simulink model "My_gfm_battery_sil_2_Exciter_Dis"  (R2018b)
settings: Solver=ode4  StartTime=0.0  StopTime=5  MaxStep=1e-4  RelTol=1e-3
PreLoadFcn:
  | modelDir = fileparts(get_param(bdroot,'FileName'));
  | 
  | load_system(fullfile(modelDir,'controls_element_lib.slx'));
  | load_system(fullfile(modelDir,'test_sequence_lib.slx'));
InitFcn:
  | close all;
  | clear all;
  | clc;
  | 
  | Ts_Power = 50e-6;
  | 
  | % frequency nominals
  | F_NOM = 60;
  | W_NOM = 2 * pi * F_NOM;
  | 
  | % base values relative to inverter
  | % --------------------------------
  | VLL_INV_NOM = 480;
  | P_INV_NOM = 1e6;
  | Q_INV_NOM = 0.5e6;
  | S_INV_NOM = sqrt(P_INV_NOM^2 + Q_INV_NOM^2);
  | 
  | I_INV_BASE = S_INV_NOM/(sqrt(3)*VLL_INV_NOM);
  | Z_INV_BASE = VLL_INV_NOM^2/S_INV_NOM;
  | L_INV_BASE = Z_INV_BASE / W_NOM;
  | C_INV_BASE = 1 / (Z_INV_BASE * W_NOM);
  | 
  | % nominal ratings for power system model
  | % --------------------------------------
  | INVERTER_COUNT = 100;
  | 
  | VLV_NOM = VLL_INV_NOM;
  | VMV_NOM = 35e3;
  | VHV_NOM = 230e3;
  | S_PLANT = INVERTER_COUNT * S_INV_NOM;
  | 
  | N_GSU = VHV_NOM/VMV_NOM;
  | N_MVT = VMV_NOM/VLV_NOM;
  | 
  | I_LV_BASE = S_PLANT/(sqrt(3)*VLV_NOM);
  | I_MV_BASE = S_PLANT/(sqrt(3)*VMV_NOM);
  | I_HV_BASE = S_PLANT/(sqrt(3)*VHV_NOM);
  | 
  | Z_LV_BASE = VLV_NOM^2/S_PLANT;
  | Z_MV_BASE = VMV_NOM^2/S_PLANT;
  | Z_HV_BASE = VHV_NOM^2/S_PLANT;
  | 
  | L_LV_BASE = Z_LV_BASE / W_NOM;
  | L_MV_BASE = Z_MV_BASE / W_NOM;
  | L_HV_BASE = Z_HV_BASE / W_NOM;
  | C_LV_BASE = 1 / (Z_LV_BASE * W_NOM);
  | C_MV_BASE = 1 / (Z_MV_BASE * W_NOM);
  | C_HV_BASE = 1 / (Z_HV_BASE * W_NOM);
undefined symbols (not defined in the file): DiscIntNeverNeededParam, j
libraries: simulink x27, test_sequence_lib x10, controls_element_lib x3
(part 4 of 5)

== system My_gfm_battery_sil_2_Exciter_Dis/My Inverter Controller /My_circuit_controls_A1/LPF1 ==
  note: Forward integrator
  in : Inport
  Constant2 : Constant  Value=Ts
  Constant3 : Constant  Value=OmegaUp
  Constant4 : Constant  Value=OmegaDn
  Constant9 : Constant  Value=1/20000
  Delay : Delay  DelayLength=1  InitialCondition=0
  Gain : Gain  Gain=1/5
  Math Function : Math  Operator=reciprocal  SaturateOnIntegerOverflow=on
  MinMax : MinMax  Function=max  Inputs=2
  MinMax1 : MinMax  Inputs=2
  MinMax2 : MinMax  Inputs=2
  Product : Product
  Product1 : Product
  Product2 : Product
  Saturation : Saturate  UpperLimit=inf  LowerLimit=0
  Saturation1 : Saturate  UpperLimit=0  LowerLimit=-inf
  Sum : Sum  Inputs=|++
  Sum1 : Sum  Inputs=|++
  Sum4 : Sum  Inputs=|+-
  out : Outport  VectorParamsAs1DForOutWhenUnconnected=on
  wires:
  Delay/1 -> out/1, Sum4/2, Sum/2
  in/1 -> Sum4/1
  Sum4/1 -> Product2/1, Product1/2
  Sum/1 -> Delay/1
  Saturation/1 -> Sum1/1
  Saturation1/1 -> Sum1/2
  Sum1/1 -> Product/2
  Product/1 -> Sum/1
  [Ts] -> Product/1
  [OmegaUp] -> Product1/1
  [OmegaDn] -> Product2/2
  Constant2/1 -> MinMax/1
  MinMax/1 -> [Ts]
  Constant9/1 -> MinMax/2
  MinMax1/1 -> [OmegaUp]
  MinMax2/1 -> [OmegaDn]
  [Ts] -> Math Function/1
  Math Function/1 -> Gain/1
  Gain/1 -> MinMax1/2, MinMax2/1
  Constant3/1 -> MinMax1/1
  Constant4/1 -> MinMax2/2
  Product1/1 -> Saturation/1
  Product2/1 -> Saturation1/1

== system My_gfm_battery_sil_2_Exciter_Dis/My Inverter Controller /My_circuit_controls_A1/LPF2 ==
  1 : Inport
  Gain2 : Gain  Gain=1/20e-6
  Integrator : Integrator
  Sum4 : Sum  Inputs=|+-
  Out1 : Outport  VectorParamsAs1DForOutWhenUnconnected=on
  wires:
  Sum4/1 -> Gain2/1
  1/1 -> Sum4/1
  Integrator/1 -> Out1/1, Sum4/2
  Gain2/1 -> Integrator/1

== system My_gfm_battery_sil_2_Exciter_Dis/My Inverter Controller /My_circuit_controls_A1/LPF3 ==
  note: Forward integrator
  in : Inport
  Constant2 : Constant  Value=Ts
  Constant3 : Constant  Value=OmegaUp
  Constant4 : Constant  Value=OmegaDn
  Constant9 : Constant  Value=1/20000
  Delay : Delay  DelayLength=1  InitialCondition=0
  Gain : Gain  Gain=1/5
  Math Function : Math  Operator=reciprocal  SaturateOnIntegerOverflow=on
  MinMax : MinMax  Function=max  Inputs=2
  MinMax1 : MinMax  Inputs=2
  MinMax2 : MinMax  Inputs=2
  Product : Product
  Product1 : Product
  Product2 : Product
  Saturation : Saturate  UpperLimit=inf  LowerLimit=0
  Saturation1 : Saturate  UpperLimit=0  LowerLimit=-inf
  Sum : Sum  Inputs=|++
  Sum1 : Sum  Inputs=|++
  Sum4 : Sum  Inputs=|+-
  out : Outport  VectorParamsAs1DForOutWhenUnconnected=on
  wires:
  Delay/1 -> out/1, Sum4/2, Sum/2
  in/1 -> Sum4/1
  Sum4/1 -> Product2/1, Product1/2
  Sum/1 -> Delay/1
  Saturation/1 -> Sum1/1
  Saturation1/1 -> Sum1/2
  Sum1/1 -> Product/2
  Product/1 -> Sum/1
  [Ts] -> Product/1
  [OmegaUp] -> Product1/1
  [OmegaDn] -> Product2/2
  Constant2/1 -> MinMax/1
  MinMax/1 -> [Ts]
  Constant9/1 -> MinMax/2
  MinMax1/1 -> [OmegaUp]
  MinMax2/1 -> [OmegaDn]
  [Ts] -> Math Function/1
  Math Function/1 -> Gain/1
  Gain/1 -> MinMax1/2, MinMax2/1
  Constant3/1 -> MinMax1/1
  Constant4/1 -> MinMax2/2
  Product1/1 -> Saturation/1
  Product2/1 -> Saturation1/1

== system My_gfm_battery_sil_2_Exciter_Dis/My Inverter Controller /My_circuit_controls_A1/LPF4 ==
  note: Forward integrator
  in : Inport
  Constant2 : Constant  Value=Ts
  Constant3 : Constant  Value=OmegaUp
  Constant4 : Constant  Value=OmegaDn
  Constant9 : Constant  Value=1/20000
  Delay : Delay  DelayLength=1  InitialCondition=0
  Gain : Gain  Gain=1/5
  Math Function : Math  Operator=reciprocal  SaturateOnIntegerOverflow=on
  MinMax : MinMax  Function=max  Inputs=2
  MinMax1 : MinMax  Inputs=2
  MinMax2 : MinMax  Inputs=2
  Product : Product
  Product1 : Product
  Product2 : Product
  Saturation : Saturate  UpperLimit=inf  LowerLimit=0
  Saturation1 : Saturate  UpperLimit=0  LowerLimit=-inf
  Sum : Sum  Inputs=|++
  Sum1 : Sum  Inputs=|++
  Sum4 : Sum  Inputs=|+-
  out : Outport  VectorParamsAs1DForOutWhenUnconnected=on
  wires:
  Delay/1 -> out/1, Sum4/2, Sum/2
  in/1 -> Sum4/1
  Sum4/1 -> Product2/1, Product1/2
  Sum/1 -> Delay/1
  Saturation/1 -> Sum1/1
  Saturation1/1 -> Sum1/2
  Sum1/1 -> Product/2
  Product/1 -> Sum/1
  [Ts] -> Product/1
  [OmegaUp] -> Product1/1
  [OmegaDn] -> Product2/2
  Constant2/1 -> MinMax/1
  MinMax/1 -> [Ts]
  Constant9/1 -> MinMax/2
  MinMax1/1 -> [OmegaUp]
  MinMax2/1 -> [OmegaDn]
  [Ts] -> Math Function/1
  Math Function/1 -> Gain/1
  Gain/1 -> MinMax1/2, MinMax2/1
  Constant3/1 -> MinMax1/1
  Constant4/1 -> MinMax2/2
  Product1/1 -> Saturation/1
  Product2/1 -> Saturation1/1

== system My_gfm_battery_sil_2_Exciter_Dis/My Inverter Controller /My_circuit_controls_A1/SOGI ==
  in : Inport
  f : Inport  Port=2
  Constant2 : Constant  Value=Ts
  Constant9 : Constant  Value=1/20000
  Gain : Gain
  Gain2 : Gain  Gain=2*pi
  Integrator1 : Subsystem
  Integrator3 : Subsystem
  MinMax : MinMax  Function=max  Inputs=2
  Product : Product
  Product2 : Product
  Sum : Sum  Inputs=|+-
  Sum1 : Sum  Inputs=|+-
  Notched : Outport  VectorParamsAs1DForOutWhenUnconnected=on
  BandPassed : Outport  Port=2  VectorParamsAs1DForOutWhenUnconnected=on
  wires:
  f/1 -> Gain2/1
  in/1 -> Sum1/1
  Integrator1/1(Out) -> Product2/1
  Gain/1 -> Sum1/2
  Sum1/1 -> Notched/1, Sum/1
  Integrator3/1(Out) -> Gain/1, BandPassed/1, Integrator1/1(In)
  Gain2/1 -> Product2/2, Product/2
  Sum/1 -> Product/1
  Product2/1 -> Sum/2
  [Ts] -> Integrator3/2(Ts)
  Product/1 -> Integrator3/1(In)
  [Ts] -> Integrator1/2(Ts)
  MinMax/1 -> [Ts]
  Constant2/1 -> MinMax/1
  Constant9/1 -> MinMax/2

== system My_gfm_battery_sil_2_Exciter_Dis/My Inverter Controller /My_circuit_controls_A1/virtual damper ==
  v : Inport
  Damping HPF : Subsystem  mask(High Pass Filter){Ts=1/20000, OmegaUp=1/250e-6, OmegaDn=1/250e-6}
      mask prompts: Ts "Tsample"; OmegaUp "Up Path Bandwidth"; OmegaDn "Down Path Bandwidth"
      mask help: Min. Tsample is 1/20000; Max. Omega is 0.2/Ts
      mask DialogControl Container2 Prompt: Parameters
  g_damp : Gain  Gain=1/(0.8*Z_INV_BASE)
  i_damp : Outport  VectorParamsAs1DForOutWhenUnconnected=on
  wires:
  g_damp/1 -> i_damp/1
  v/1 -> Damping HPF/1(in)
  Damping HPF/1(out) -> g_damp/1

== system My_gfm_battery_sil_2_Exciter_Dis/My Inverter Controller /My_circuit_controls_A2/LPF ==
  1 : Inport
  Gain2 : Gain  Gain=1/20e-6
  Integrator : Integrator
  Sum4 : Sum  Inputs=|+-
  Out1 : Outport  VectorParamsAs1DForOutWhenUnconnected=on
  wires:
  Gain2/1 -> Integrator/1
  Integrator/1 -> Sum4/2, Out1/1
  1/1 -> Sum4/1
  Sum4/1 -> Gain2/1

== system My_gfm_battery_sil_2_Exciter_Dis/My Inverter Controller /My_circuit_controls_A2/LPF1 ==
  1 : Inport
  Gain2 : Gain  Gain=1/20e-6
  Integrator : Integrator
  Sum4 : Sum  Inputs=|+-
  Out1 : Outport  VectorParamsAs1DForOutWhenUnconnected=on
  wires:
  Gain2/1 -> Integrator/1
  Integrator/1 -> Sum4/2, Out1/1
  1/1 -> Sum4/1
  Sum4/1 -> Gain2/1

== system My_gfm_battery_sil_2_Exciter_Dis/My Inverter Controller /My_circuit_controls_A2/LPF2 ==
  1 : Inport
  Gain2 : Gain  Gain=1/20e-6
  Integrator : Integrator
  Sum4 : Sum  Inputs=|+-
  Out1 : Outport  VectorParamsAs1DForOutWhenUnconnected=on
  wires:
  Sum4/1 -> Gain2/1
  1/1 -> Sum4/1
  Integrator/1 -> Out1/1, Sum4/2
  Gain2/1 -> Integrator/1

== system My_gfm_battery_sil_2_Exciter_Dis/My Inverter Controller /My_circuit_controls_A2/LPF3 ==
  1 : Inport
  Gain2 : Gain  Gain=1/500e-6
  Integrator : Integrator
  Sum4 : Sum  Inputs=|+-
  Out1 : Outport  VectorParamsAs1DForOutWhenUnconnected=on
  wires:
  Gain2/1 -> Integrator/1
  Integrator/1 -> Sum4/2, Out1/1
  1/1 -> Sum4/1
  Sum4/1 -> Gain2/1

== system My_gfm_battery_sil_2_Exciter_Dis/My Inverter Controller /My_circuit_controls_A2/LPF4 ==
  1 : Inport
  Gain2 : Gain  Gain=1/20e-6
  Integrator : Integrator
  Sum4 : Sum  Inputs=|+-
  Out1 : Outport  VectorParamsAs1DForOutWhenUnconnected=on
  wires:
  Gain2/1 -> Integrator/1
  Integrator/1 -> Sum4/2, Out1/1
  1/1 -> Sum4/1
  Sum4/1 -> Gain2/1

== system My_gfm_battery_sil_2_Exciter_Dis/My Inverter Controller /My_circuit_controls_A2/SOGI_BPF ==
  in : Inport
  f : Inport  Port=2
  Gain : Gain
  Gain2 : Gain  Gain=2*pi
  Integrator : Integrator
  Integrator1 : Integrator
  Product : Product
  Product2 : Product
  Sum : Sum  Inputs=|+-
  Sum1 : Sum  Inputs=|+-
  Notched : Outport  VectorParamsAs1DForOutWhenUnconnected=on
  wires:
  f/1 -> Gain2/1
  in/1 -> Sum1/1
  Product/1 -> Integrator/1
  Integrator1/1 -> Product2/1
  Gain/1 -> Sum1/2
  Sum1/1 -> Notched/1, Sum/1
  Integrator/1 -> Integrator1/1, Gain/1
  Gain2/1 -> Product2/2, Product/2
  Sum/1 -> Product/1
  Product2/1 -> Sum/2

== system My_gfm_battery_sil_2_Exciter_Dis/My Inverter Controller /My_circuit_controls_A2/virtual damper ==
  v : Inport
  1/tau_damp : Gain  Gain=1/250e-6
  Integrator : Integrator
  Sum : Sum  Inputs=|+-
  g_damp : Gain  Gain=1/(0.8*Z_INV_BASE)
  i_damp : Outport  VectorParamsAs1DForOutWhenUnconnected=on
  wires:
  g_damp/1 -> i_damp/1
  Sum/1 -> g_damp/1, 1/tau_damp/1
  v/1 -> Sum/1
  1/tau_damp/1 -> Integrator/1
  Integrator/1 -> Sum/2

== system My_gfm_battery_sil_2_Exciter_Dis/My Inverter Controller /My_circuit_controls_A3/LPF ==
  1 : Inport
  Gain2 : Gain  Gain=1/20e-6
  Integrator : Integrator
  Sum4 : Sum  Inputs=|+-
  Out1 : Outport  VectorParamsAs1DForOutWhenUnconnected=on
  wires:
  Gain2/1 -> Integrator/1
  Integrator/1 -> Sum4/2, Out1/1
  1/1 -> Sum4/1
  Sum4/1 -> Gain2/1

== system My_gfm_battery_sil_2_Exciter_Dis/My Inverter Controller /My_circuit_controls_A3/LPF1 ==
  1 : Inport
  Gain2 : Gain  Gain=1/20e-6
  Integrator : Integrator
  Sum4 : Sum  Inputs=|+-
  Out1 : Outport  VectorParamsAs1DForOutWhenUnconnected=on
  wires:
  Gain2/1 -> Integrator/1
  Integrator/1 -> Sum4/2, Out1/1
  1/1 -> Sum4/1
  Sum4/1 -> Gain2/1

== system My_gfm_battery_sil_2_Exciter_Dis/My Inverter Controller /My_circuit_controls_A3/LPF2 ==
  1 : Inport
  Gain2 : Gain  Gain=1/20e-6
  Integrator : Integrator
  Sum4 : Sum  Inputs=|+-
  Out1 : Outport  VectorParamsAs1DForOutWhenUnconnected=on
  wires:
  Sum4/1 -> Gain2/1
  1/1 -> Sum4/1
  Integrator/1 -> Out1/1, Sum4/2
  Gain2/1 -> Integrator/1

== system My_gfm_battery_sil_2_Exciter_Dis/My Inverter Controller /My_circuit_controls_A3/LPF3 ==
  note: Forward integrator
  in : Inport
  Constant2 : Constant  Value=Ts
  Constant3 : Constant  Value=OmegaUp
  Constant4 : Constant  Value=OmegaDn
  Constant9 : Constant  Value=1/20000
  Delay : Delay  DelayLength=1  InitialCondition=0
  Gain : Gain  Gain=1/5
  Math Function : Math  Operator=reciprocal  SaturateOnIntegerOverflow=on
  MinMax : MinMax  Function=max  Inputs=2
  MinMax1 : MinMax  Inputs=2
  MinMax2 : MinMax  Inputs=2
  Product : Product
  Product1 : Product
  Product2 : Product
  Saturation : Saturate  UpperLimit=inf  LowerLimit=0
  Saturation1 : Saturate  UpperLimit=0  LowerLimit=-inf
  Sum : Sum  Inputs=|++
  Sum1 : Sum  Inputs=|++
  Sum4 : Sum  Inputs=|+-
  out : Outport  VectorParamsAs1DForOutWhenUnconnected=on
  wires:
  Delay/1 -> out/1, Sum4/2, Sum/2
  in/1 -> Sum4/1
  Sum4/1 -> Product2/1, Product1/2
  Sum/1 -> Delay/1
  Saturation/1 -> Sum1/1
  Saturation1/1 -> Sum1/2
  Sum1/1 -> Product/2
  Product/1 -> Sum/1
  [Ts] -> Product/1
  [OmegaUp] -> Product1/1
  [OmegaDn] -> Product2/2
  Constant2/1 -> MinMax/1
  MinMax/1 -> [Ts]
  Constant9/1 -> MinMax/2
  MinMax1/1 -> [OmegaUp]
  MinMax2/1 -> [OmegaDn]
  [Ts] -> Math Function/1
  Math Function/1 -> Gain/1
  Gain/1 -> MinMax1/2, MinMax2/1
  Constant3/1 -> MinMax1/1
  Constant4/1 -> MinMax2/2
  Product1/1 -> Saturation/1
  Product2/1 -> Saturation1/1

== system My_gfm_battery_sil_2_Exciter_Dis/My Inverter Controller /My_circuit_controls_A3/LPF4 ==
  note: Forward integrator
  in : Inport
  Constant2 : Constant  Value=Ts
  Constant3 : Constant  Value=OmegaUp
  Constant4 : Constant  Value=OmegaDn
  Constant9 : Constant  Value=1/20000
  Delay : Delay  DelayLength=1  InitialCondition=0
  Gain : Gain  Gain=1/5
  Math Function : Math  Operator=reciprocal  SaturateOnIntegerOverflow=on
  MinMax : MinMax  Function=max  Inputs=2
  MinMax1 : MinMax  Inputs=2
  MinMax2 : MinMax  Inputs=2
  Product : Product
  Product1 : Product
  Product2 : Product
  Saturation : Saturate  UpperLimit=inf  LowerLimit=0
  Saturation1 : Saturate  UpperLimit=0  LowerLimit=-inf
  Sum : Sum  Inputs=|++
  Sum1 : Sum  Inputs=|++
  Sum4 : Sum  Inputs=|+-
  out : Outport  VectorParamsAs1DForOutWhenUnconnected=on
  wires:
  Delay/1 -> out/1, Sum4/2, Sum/2
  in/1 -> Sum4/1
  Sum4/1 -> Product2/1, Product1/2
  Sum/1 -> Delay/1
  Saturation/1 -> Sum1/1
  Saturation1/1 -> Sum1/2
  Sum1/1 -> Product/2
  Product/1 -> Sum/1
  [Ts] -> Product/1
  [OmegaUp] -> Product1/1
  [OmegaDn] -> Product2/2
  Constant2/1 -> MinMax/1
  MinMax/1 -> [Ts]
  Constant9/1 -> MinMax/2
  MinMax1/1 -> [OmegaUp]
  MinMax2/1 -> [OmegaDn]
  [Ts] -> Math Function/1
  Math Function/1 -> Gain/1
  Gain/1 -> MinMax1/2, MinMax2/1
  Constant3/1 -> MinMax1/1
  Constant4/1 -> MinMax2/2
  Product1/1 -> Saturation/1
  Product2/1 -> Saturation1/1

== system My_gfm_battery_sil_2_Exciter_Dis/My Inverter Controller /My_circuit_controls_A3/SOGI_BPF ==
  in : Inport
  f : Inport  Port=2
  Discrete-Time Integrator : DiscreteIntegrator  SampleTime=1/20000  ICPrevOutput=DiscIntNeverNeededParam  ICPrevScaledInput=DiscIntNeverNeededParam
  Discrete-Time Integrator1 : DiscreteIntegrator  SampleTime=1/20000  ICPrevOutput=DiscIntNeverNeededParam  ICPrevScaledInput=DiscIntNeverNeededParam
  Gain : Gain
  Gain2 : Gain  Gain=2*pi
  Product : Product
  Product2 : Product
  Sum : Sum  Inputs=|+-
  Sum1 : Sum  Inputs=|+-
  Notched : Outport  VectorParamsAs1DForOutWhenUnconnected=on
  wires:
  f/1 -> Gain2/1
  in/1 -> Sum1/1
  Product/1 -> Discrete-Time Integrator/1
  Discrete-Time Integrator/1 -> Discrete-Time Integrator1/1, Gain/1
  Gain/1 -> Sum1/2
  Sum1/1 -> Notched/1, Sum/1
  Gain2/1 -> Product2/2, Product/2
  Sum/1 -> Product/1
  Product2/1 -> Sum/2
  Discrete-Time Integrator1/1 -> Product2/1

== system My_gfm_battery_sil_2_Exciter_Dis/My Inverter Controller /My_circuit_controls_A3/virtual damper ==
  v : Inport
  Damping HPF : Subsystem  mask(High Pass Filter){Ts=1/20000, OmegaUp=1/250e-6, OmegaDn=1/250e-6}
      mask prompts: Ts "Tsample"; OmegaUp "Up Path Bandwidth"; OmegaDn "Down Path Bandwidth"
      mask help: Min. Tsample is 1/20000; Max. Omega is 0.2/Ts
      mask DialogControl Container2 Prompt: Parameters
  g_damp : Gain  Gain=1/(0.8*Z_INV_BASE)
  i_damp : Outport  VectorParamsAs1DForOutWhenUnconnected=on
  wires:
  g_damp/1 -> i_damp/1
  v/1 -> Damping HPF/1(in)
  Damping HPF/1(out) -> g_damp/1

== system My_gfm_battery_sil_2_Exciter_Dis/My Inverter Controller /My_circuit_controls_A4/LPF1 ==
  note: Forward integrator
  in : Inport
  Constant2 : Constant  Value=Ts
  Constant3 : Constant  Value=OmegaUp
  Constant4 : Constant  Value=OmegaDn
  Constant9 : Constant  Value=1/20000
  Delay : Delay  DelayLength=1  InitialCondition=0
  Gain : Gain  Gain=1/5
  Math Function : Math  Operator=reciprocal  SaturateOnIntegerOverflow=on
  MinMax : MinMax  Function=max  Inputs=2
  MinMax1 : MinMax  Inputs=2
  MinMax2 : MinMax  Inputs=2
  Product : Product
  Product1 : Product
  Product2 : Product
  Saturation : Saturate  UpperLimit=inf  LowerLimit=0
  Saturation1 : Saturate  UpperLimit=0  LowerLimit=-inf
  Sum : Sum  Inputs=|++
  Sum1 : Sum  Inputs=|++
  Sum4 : Sum  Inputs=|+-
  out : Outport  VectorParamsAs1DForOutWhenUnconnected=on
  wires:
  Delay/1 -> out/1, Sum4/2, Sum/2
  in/1 -> Sum4/1
  Sum4/1 -> Product2/1, Product1/2
  Sum/1 -> Delay/1
  Saturation/1 -> Sum1/1
  Saturation1/1 -> Sum1/2
  Sum1/1 -> Product/2
  Product/1 -> Sum/1
  [Ts] -> Product/1
  [OmegaUp] -> Product1/1
  [OmegaDn] -> Product2/2
  Constant2/1 -> MinMax/1
  MinMax/1 -> [Ts]
  Constant9/1 -> MinMax/2
  MinMax1/1 -> [OmegaUp]
  MinMax2/1 -> [OmegaDn]
  [Ts] -> Math Function/1
  Math Function/1 -> Gain/1
  Gain/1 -> MinMax1/2, MinMax2/1
  Constant3/1 -> MinMax1/1
  Constant4/1 -> MinMax2/2
  Product1/1 -> Saturation/1
  Product2/1 -> Saturation1/1

== system My_gfm_battery_sil_2_Exciter_Dis/My Inverter Controller /My_circuit_controls_A4/LPF2 ==
  1 : Inport
  Gain2 : Gain  Gain=1/20e-6
  Integrator : Integrator
  Sum4 : Sum  Inputs=|+-
  Out1 : Outport  VectorParamsAs1DForOutWhenUnconnected=on
  wires:
  Sum4/1 -> Gain2/1
  1/1 -> Sum4/1
  Integrator/1 -> Out1/1, Sum4/2
  Gain2/1 -> Integrator/1

== system My_gfm_battery_sil_2_Exciter_Dis/My Inverter Controller /My_circuit_controls_A4/LPF3 ==
  note: Forward integrator
  in : Inport
  Constant2 : Constant  Value=Ts
  Constant3 : Constant  Value=OmegaUp
  Constant4 : Constant  Value=OmegaDn
  Constant9 : Constant  Value=1/20000
  Delay : Delay  DelayLength=1  InitialCondition=0
  Gain : Gain  Gain=1/5
  Math Function : Math  Operator=reciprocal  SaturateOnIntegerOverflow=on
  MinMax : MinMax  Function=max  Inputs=2
  MinMax1 : MinMax  Inputs=2
  MinMax2 : MinMax  Inputs=2
  Product : Product
  Product1 : Product
  Product2 : Product
  Saturation : Saturate  UpperLimit=inf  LowerLimit=0
  Saturation1 : Saturate  UpperLimit=0  LowerLimit=-inf
  Sum : Sum  Inputs=|++
  Sum1 : Sum  Inputs=|++
  Sum4 : Sum  Inputs=|+-
  out : Outport  VectorParamsAs1DForOutWhenUnconnected=on
  wires:
  Delay/1 -> out/1, Sum4/2, Sum/2
  in/1 -> Sum4/1
  Sum4/1 -> Product2/1, Product1/2
  Sum/1 -> Delay/1
  Saturation/1 -> Sum1/1
  Saturation1/1 -> Sum1/2
  Sum1/1 -> Product/2
  Product/1 -> Sum/1
  [Ts] -> Product/1
  [OmegaUp] -> Product1/1
  [OmegaDn] -> Product2/2
  Constant2/1 -> MinMax/1
  MinMax/1 -> [Ts]
  Constant9/1 -> MinMax/2
  MinMax1/1 -> [OmegaUp]
  MinMax2/1 -> [OmegaDn]
  [Ts] -> Math Function/1
  Math Function/1 -> Gain/1
  Gain/1 -> MinMax1/2, MinMax2/1
  Constant3/1 -> MinMax1/1
  Constant4/1 -> MinMax2/2
  Product1/1 -> Saturation/1
  Product2/1 -> Saturation1/1

== system My_gfm_battery_sil_2_Exciter_Dis/My Inverter Controller /My_circuit_controls_A4/LPF4 ==
  note: Forward integrator
  in : Inport
  Constant2 : Constant  Value=Ts
  Constant3 : Constant  Value=OmegaUp
  Constant4 : Constant  Value=OmegaDn
  Constant9 : Constant  Value=1/20000
  Delay : Delay  DelayLength=1  InitialCondition=0
  Gain : Gain  Gain=1/5
  Math Function : Math  Operator=reciprocal  SaturateOnIntegerOverflow=on
  MinMax : MinMax  Function=max  Inputs=2
  MinMax1 : MinMax  Inputs=2
  MinMax2 : MinMax  Inputs=2
  Product : Product
  Product1 : Product
  Product2 : Product
  Saturation : Saturate  UpperLimit=inf  LowerLimit=0
  Saturation1 : Saturate  UpperLimit=0  LowerLimit=-inf
  Sum : Sum  Inputs=|++
  Sum1 : Sum  Inputs=|++
  Sum4 : Sum  Inputs=|+-
  out : Outport  VectorParamsAs1DForOutWhenUnconnected=on
  wires:
  Delay/1 -> out/1, Sum4/2, Sum/2
  in/1 -> Sum4/1
  Sum4/1 -> Product2/1, Product1/2
  Sum/1 -> Delay/1
  Saturation/1 -> Sum1/1
  Saturation1/1 -> Sum1/2
  Sum1/1 -> Product/2
  Product/1 -> Sum/1
  [Ts] -> Product/1
  [OmegaUp] -> Product1/1
  [OmegaDn] -> Product2/2
  Constant2/1 -> MinMax/1
  MinMax/1 -> [Ts]
  Constant9/1 -> MinMax/2
  MinMax1/1 -> [OmegaUp]
  MinMax2/1 -> [OmegaDn]
  [Ts] -> Math Function/1
  Math Function/1 -> Gain/1
  Gain/1 -> MinMax1/2, MinMax2/1
  Constant3/1 -> MinMax1/1
  Constant4/1 -> MinMax2/2
  Product1/1 -> Saturation/1
  Product2/1 -> Saturation1/1

== system My_gfm_battery_sil_2_Exciter_Dis/My Inverter Controller /My_circuit_controls_A4/LPF5 ==
  note: Forward integrator
  in : Inport
  Constant2 : Constant  Value=Ts
  Constant3 : Constant  Value=OmegaUp
  Constant4 : Constant  Value=OmegaDn
  Constant9 : Constant  Value=1/20000
  Delay : Delay  DelayLength=1  InitialCondition=0
  Gain : Gain  Gain=1/5
  Math Function : Math  Operator=reciprocal  SaturateOnIntegerOverflow=on
  MinMax : MinMax  Function=max  Inputs=2
  MinMax1 : MinMax  Inputs=2
  MinMax2 : MinMax  Inputs=2
  Product : Product
  Product1 : Product
  Product2 : Product
  Saturation : Saturate  UpperLimit=inf  LowerLimit=0
  Saturation1 : Saturate  UpperLimit=0  LowerLimit=-inf
  Sum : Sum  Inputs=|++
  Sum1 : Sum  Inputs=|++
  Sum4 : Sum  Inputs=|+-
  out : Outport  VectorParamsAs1DForOutWhenUnconnected=on
  wires:
  Delay/1 -> out/1, Sum4/2, Sum/2
  in/1 -> Sum4/1
  Sum4/1 -> Product2/1, Product1/2
  Sum/1 -> Delay/1
  Saturation/1 -> Sum1/1
  Saturation1/1 -> Sum1/2
  Sum1/1 -> Product/2
  Product/1 -> Sum/1
  [Ts] -> Product/1
  [OmegaUp] -> Product1/1
  [OmegaDn] -> Product2/2
  Constant2/1 -> MinMax/1
  MinMax/1 -> [Ts]
  Constant9/1 -> MinMax/2
  MinMax1/1 -> [OmegaUp]
  MinMax2/1 -> [OmegaDn]
  [Ts] -> Math Function/1
  Math Function/1 -> Gain/1
  Gain/1 -> MinMax1/2, MinMax2/1
  Constant3/1 -> MinMax1/1
  Constant4/1 -> MinMax2/2
  Product1/1 -> Saturation/1
  Product2/1 -> Saturation1/1

== system My_gfm_battery_sil_2_Exciter_Dis/My Inverter Controller /My_circuit_controls_A4/SOGI ==
  in : Inport
  f : Inport  Port=2
  Constant2 : Constant  Value=Ts
  Constant9 : Constant  Value=1/20000
  Gain : Gain
  Gain2 : Gain  Gain=2*pi
  Integrator1 : Subsystem
  Integrator3 : Subsystem
  MinMax : MinMax  Function=max  Inputs=2
  Product : Product
  Product2 : Product
  Sum : Sum  Inputs=|+-
  Sum1 : Sum  Inputs=|+-
  Notched : Outport  VectorParamsAs1DForOutWhenUnconnected=on
  BandPassed : Outport  Port=2  VectorParamsAs1DForOutWhenUnconnected=on
  wires:
  f/1 -> Gain2/1
  in/1 -> Sum1/1
  Integrator1/1(Out) -> Product2/1
  Gain/1 -> Sum1/2
  Sum1/1 -> Notched/1, Sum/1
  Integrator3/1(Out) -> Gain/1, BandPassed/1, Integrator1/1(In)
  Gain2/1 -> Product2/2, Product/2
  Sum/1 -> Product/1
  Product2/1 -> Sum/2
  [Ts] -> Integrator3/2(Ts)
  Product/1 -> Integrator3/1(In)
  [Ts] -> Integrator1/2(Ts)
  MinMax/1 -> [Ts]
  Constant2/1 -> MinMax/1
  Constant9/1 -> MinMax/2

== system My_gfm_battery_sil_2_Exciter_Dis/My Inverter Controller /My_circuit_controls_A4/virtual damper ==
  v : Inport
  Damping HPF : Subsystem  mask(High Pass Filter){Ts=1/20000, OmegaUp=1/250e-6, OmegaDn=1/250e-6}
      mask prompts: Ts "Tsample"; OmegaUp "Up Path Bandwidth"; OmegaDn "Down Path Bandwidth"
      mask help: Min. Tsample is 1/20000; Max. Omega is 0.2/Ts
      mask DialogControl Container2 Prompt: Parameters
  g_damp : Gain  Gain=1/(0.8*Z_INV_BASE)
  i_damp : Outport  VectorParamsAs1DForOutWhenUnconnected=on
  wires:
  g_damp/1 -> i_damp/1
  v/1 -> Damping HPF/1(in)
  Damping HPF/1(out) -> g_damp/1

== system My_gfm_battery_sil_2_Exciter_Dis/My Inverter Controller /My_currentLimiting_B/Current_foldback1 ==
  V[3]_pu : Inport
  Vmax : Inport  Port=2
  Abs1 : Abs
  Constant1 : Constant
  Gain : Gain  Gain=5
  "LPF " : Subsystem
  Max : MinMax  Function=max
  Saturation : Saturate  UpperLimit=1  LowerLimit=0.05
  Scope1 : Scope  NumInputPorts=3
  Sum1 : Sum  Inputs=|+-
  Sum2 : Sum  Inputs=|++
  Transfer Fcn : TransferFcn  Denominator=[0.01 1]
  limit_pu : Outport  VectorParamsAs1DForOutWhenUnconnected=on
  wires:
  "LPF "/1(Out) -> Gain/1
  V[3]_pu/1 -> Abs1/1
  Sum2/1 -> Saturation/1
  Constant1/1 -> Sum2/2
  Vmax/1 -> Scope1/1, Sum1/1
  Saturation/1 -> limit_pu/1
  Abs1/1 -> Max/1
  Max/1 -> Sum1/2, Scope1/3
  Sum1/1 -> "LPF "/1(In), Scope1/2
  Gain/1 -> Sum2/1

== system My_gfm_battery_sil_2_Exciter_Dis/My Inverter Controller /My_currentLimiting_B/RMS_Analyzer ==
  in : Inport
  Gain : Gain  Gain=1/0.02
  Integrator : Integrator
  Sqrt : Sqrt  SaturateOnIntegerOverflow=on
  Square : Math  Operator=square  SaturateOnIntegerOverflow=on
  Sum : Sum  Inputs=|+-
  RMS : Outport  VectorParamsAs1DForOutWhenUnconnected=on
  wires:
  Square/1 -> Sum/1
  in/1 -> Square/1
  Gain/1 -> Integrator/1
  Sum/1 -> Gain/1
  Integrator/1 -> Sum/2, Sqrt/1
  Sqrt/1 -> RMS/1

== system My_gfm_battery_sil_2_Exciter_Dis/My Inverter Controller /My_currentLimiting_B/RMS_Analyzer1 ==
  in : Inport
  Gain : Gain  Gain=1/0.02
  Integrator : Integrator
  Sqrt : Sqrt  SaturateOnIntegerOverflow=on
  Square : Math  Operator=square  SaturateOnIntegerOverflow=on
  Sum : Sum  Inputs=|+-
  RMS : Outport  VectorParamsAs1DForOutWhenUnconnected=on
  wires:
  Square/1 -> Sum/1
  in/1 -> Square/1
  Gain/1 -> Integrator/1
  Sum/1 -> Gain/1
  Integrator/1 -> Sum/2, Sqrt/1
  Sqrt/1 -> RMS/1

== system My_gfm_battery_sil_2_Exciter_Dis/My Inverter Controller /My_currentLimiting_B/SOGI_BPF ==
  in : Inport
  f : Inport  Port=2
  Gain : Gain
  Gain2 : Gain  Gain=2*pi
  Integrator : Integrator
  Integrator1 : Integrator
  Product : Product
  Product2 : Product
  Sum : Sum  Inputs=|+-
  Sum1 : Sum  Inputs=|+-
  bpf : Outport  VectorParamsAs1DForOutWhenUnconnected=on
  wires:
  f/1 -> Gain2/1
  in/1 -> Sum1/1
  Product/1 -> Integrator/1
  Integrator1/1 -> Product2/1
  Gain/1 -> Sum1/2
  Sum1/1 -> Sum/1
  Integrator/1 -> Integrator1/1, Gain/1, bpf/1
  Gain2/1 -> Product2/2, Product/2
  Sum/1 -> Product/1
  Product2/1 -> Sum/2

== system My_gfm_battery_sil_2_Exciter_Dis/My Inverter Controller /My_currentLimiting_B/estimate_excess ==
  note: why?
  note: Iabc rms
  Ilimit : Inport
  I[3] : Inport  Port=2
  Abs1 : Abs
  Constant : Constant
  Max : MinMax  Function=max
  Min : MinMax  Function=max  Inputs=2
  Product1 : Product  Inputs=*/
  Scope11 : Scope  NumInputPorts=4
  Sum : Sum  Inputs=|+-
  excess_fraction : Outport  VectorParamsAs1DForOutWhenUnconnected=on
  wires:
  Sum/1 -> excess_fraction/1
  Constant/1 -> Sum/1
  Product1/1 -> Sum/2  "scale_factor"
  Max/1 -> Scope11/3, Min/2  "max_Iph"
  Ilimit/1 -> Scope11/1, Product1/1, Min/1  "Irms_limit"
  Abs1/1 -> Max/1
  I[3]/1 -> Scope11/4, Abs1/1
  Min/1 -> Scope11/2, Product1/2

== system My_gfm_battery_sil_2_Exciter_Dis/My Inverter Controller /My_currentLimiting_B/soft_saturation ==
  note: 1-e(-dx/H)
  note: dX
  note: dX/Xau
  note: -1+e(-dx/H)
  note: H*[1-e(-dx/H)] + H*[-1+e(-dx/H)]
  in : Inport
  Constant : Constant
  Constant1 : Constant
  Exp : Math  SaturateOnIntegerOverflow=on
  Exp1 : Math  SaturateOnIntegerOverflow=on
  Gain : Gain  Gain=-1
  Gain1 : Gain  Gain=Xau
  Product : Product  Inputs=*/
  Sum : Sum  Inputs=|++
  Sum1 : Sum  Inputs=-+|
  Sum2 : Sum  Inputs=|+-
  Sum3 : Sum  Inputs=|+-
  Sum4 : Sum  Inputs=|++
  headroom : Gain  Gain=(hard_limit - soft_limit)
  headroom1 : Constant  Value=max(hard_limit - soft_limit, 1e-3)
  negative : Saturate  UpperLimit=0  LowerLimit=-inf
  positive : Saturate  UpperLimit=inf  LowerLimit=0
  soft_limit : Saturate  UpperLimit=soft_limit  LowerLimit=-soft_limit
  out : Outport  VectorParamsAs1DForOutWhenUnconnected=on
  wires:
  headroom1/1 -> Gain1/1
  Sum1/1 -> Product/1
  Sum2/1 -> Sum4/1
  Sum4/1 -> headroom/1
  Gain/1 -> Exp/1
  headroom/1 -> Sum/2
  Exp/1 -> Sum2/2
  positive/1 -> Gain/1
  in/1 -> soft_limit/1, Sum1/2
  Exp1/1 -> Sum3/1
  Sum/1 -> out/1
  soft_limit/1 -> Sum1/1, Sum/1
  Sum3/1 -> Sum4/2
  negative/1 -> Exp1/1
  Constant1/1 -> Sum3/2
  Product/1 -> positive/1, negative/1
  Constant/1 -> Sum2/1
  Gain1/1 -> Product/2  "Xau"

== system My_gfm_battery_sil_2_Exciter_Dis/My Inverter Controller /My_currentLimiting_B/soft_saturation1 ==
  in : Inport
  Constant : Constant
  Constant1 : Constant
  Exp : Math  SaturateOnIntegerOverflow=on
  Exp1 : Math  SaturateOnIntegerOverflow=on
  Gain : Gain  Gain=-1
  Product : Product  Inputs=*/
  Sum : Sum  Inputs=|++
  Sum1 : Sum  Inputs=-+|
  Sum2 : Sum  Inputs=|+-
  Sum3 : Sum  Inputs=|+-
  Sum4 : Sum  Inputs=|++
  headroom : Gain  Gain=(hard_limit - soft_limit)
  headroom1 : Constant  Value=max(hard_limit - soft_limit, 1e-3)
  negative : Saturate  UpperLimit=0  LowerLimit=-inf
  positive : Saturate  UpperLimit=inf  LowerLimit=0
  soft_limit : Saturate  UpperLimit=soft_limit  LowerLimit=-soft_limit
  out : Outport  VectorParamsAs1DForOutWhenUnconnected=on
  wires:
  headroom1/1 -> Product/2
  Sum1/1 -> Product/1
  Sum2/1 -> Sum4/1
  Sum4/1 -> headroom/1
  Gain/1 -> Exp/1
  headroom/1 -> Sum/2
  Exp/1 -> Sum2/2
  positive/1 -> Gain/1
  in/1 -> soft_limit/1, Sum1/2
  Exp1/1 -> Sum3/1
  Sum/1 -> out/1
  soft_limit/1 -> Sum1/1, Sum/1
  Sum3/1 -> Sum4/2
  negative/1 -> Exp1/1
  Constant1/1 -> Sum3/2
  Product/1 -> positive/1, negative/1
  Constant/1 -> Sum2/1

== system My_gfm_battery_sil_2_Exciter_Dis/My Inverter Controller /My_currentSource_A/current_modulator ==
  I_cmd : Inport
  osc : Inport  Port=2
  Complex to Real-Imag : ComplexToRealImag
  Complex to Real-Imag1 : ComplexToRealImag
  Gain : Gain  Gain=sqrt(2)
  Product1 : Product
  Product2 : Product
  Sum1 : Sum  Inputs=|+-
  i_ref : Outport  VectorParamsAs1DForOutWhenUnconnected=on
  wires:
  osc/1 -> Gain/1
  Complex to Real-Imag/1 -> Product2/2
  Product2/1 -> Sum1/1
  Sum1/1 -> i_ref/1  "i"
  Gain/1 -> Complex to Real-Imag/1
  Complex to Real-Imag/2 -> Product1/2
  Product1/1 -> Sum1/2
  I_cmd/1 -> Complex to Real-Imag1/1
  Complex to Real-Imag1/1 -> Product2/1
  Complex to Real-Imag1/2 -> Product1/1

== system My_gfm_battery_sil_2_Exciter_Dis/My Inverter Controller /My_machineModel_Other Exciter/AVR ==
  note: This limit is needed to avoid excessive currents during blackstart that cause windup in current limiting logic.. It results in a linear ramp of voltage during blackstart
  note: Using asym filter to traget long extended low voltage events, prevent it from acting during typical faults
  VRef : Inport
  Vt : Inport  Port=2
  Q : Inport  Port=3
  Gain : Gain  Gain=VllRated
  Gain3 : Gain  Gain=Qleak
  Gain4 : Gain  Gain=1/VllRated
  Gain5 : Gain  Gain=1/VllRated
  Integrator : Integrator  LimitOutput=on  UpperSaturationLimit=0.1  LowerSaturationLimit=-0.1
  LPF : Subsystem
  Min : MinMax  Inputs=2
  Saturation1 : Saturate  UpperLimit=1.1*VllRated  LowerLimit=0.90*VllRated
  Saturation2 : Saturate  UpperLimit=0.2  LowerLimit=-0.2
  Saturation3 : Saturate  UpperLimit=0.1*VllRated  LowerLimit=-0.1*VllRated
  Sum : Sum  Inputs=++|
  Sum1 : Sum  Inputs=|+-
  Sum2 : Sum  Inputs=+-|
  Sum3 : Sum  Inputs=|++
  Sum4 : Sum  Inputs=|+-
  Sum5 : Sum  Inputs=++|
  V LPF : Subsystem
  assymmetric filter : Subsystem
  ki : Gain  Gain=kiq
  kp : Gain  Gain=kpq
  kpv : Gain  Gain=Kpv
  p.u1 : Gain  Gain=1/SRated
  p.u2 : Gain  Gain=VllRated
  voltage_headroom : Constant  Value=Xs
  Vexc : Outport  VectorParamsAs1DForOutWhenUnconnected=on
  wires:
  Sum/1 -> Min/2
  voltage_headroom/1 -> Gain/1
  assymmetric filter/1(out) -> Sum/2  "Vt_conditioned"
  Vt/1 -> assymmetric filter/1(in), Gain4/1  "Vt"
  Min/1 -> Sum5/1, Gain5/1
  kpv/1 -> V LPF/1(In)
  kp/1 -> Sum3/1
  Sum5/1 -> Vexc/1
  Sum2/1 -> Saturation2/1
  Sum3/1 -> p.u2/1
  Sum4/1 -> Integrator/1
  Integrator/1 -> Sum3/2, Gain3/1
  ki/1 -> Sum4/1
  Gain3/1 -> Sum4/2
  Gain/1 -> Sum/1
  VRef/1 -> Saturation1/1  "VRef"
  Q/1 -> LPF/1(In)
  LPF/1(Out) -> p.u1/1
  p.u1/1 -> Sum1/2
  V LPF/1(Out) -> Sum1/1
  Gain4/1 -> Sum2/2
  Gain5/1 -> Sum2/1
  Saturation1/1 -> Min/1
  p.u2/1 -> Saturation3/1
  Saturation3/1 -> Sum5/2
  Saturation2/1 -> kpv/1
  Sum1/1 -> ki/1, kp/1

== system My_gfm_battery_sil_2_Exciter_Dis/My Inverter Controller /My_machineModel_Other Exciter/Exciter ==
  note: Aligning with Rotor Frame
      | cos x + j sin x
      | cos (x-120) + j (sin x -120)
      | cos (x+120) + j (sin x +120)
  note: Vb = vd * cos (x-120) - vq * sin (x-120)
  note: Peak EMFa,b,c
  note: Va = vd * cos x - vq * sin x
  note: Vq = 0
  note: Vc = vd * cos (x+120) - vq * sin (x+120)
  Vexc : Inport
  osc[3] : Inport  Port=2
  Constant : Constant  Value=0
  Gain2 : Gain  Gain=1/sqrt(3)
  LPF : Subsystem
  LPF1 : TransferFcn  Commented=on  Denominator=[1/wExciter 1]
  Real-Imag to Complex : RealImagToComplex
  modulator : Subsystem
  v_emf : Outport  VectorParamsAs1DForOutWhenUnconnected=on
  wires:
  LPF/1(Out) -> Gain2/1  "Vref_LL"
  modulator/1(ref) -> v_emf/1
  Gain2/1 -> Real-Imag to Complex/1  "Vref_LN"
  osc[3]/1 -> modulator/2(osc)
  Constant/1 -> Real-Imag to Complex/2
  Real-Imag to Complex/1 -> modulator/1(cmd)
  Vexc/1 -> LPF/1(In)

== system My_gfm_battery_sil_2_Exciter_Dis/My Inverter Controller /My_machineModel_Other Exciter/governer ==
  note: Machine enables
  note: RMS LL
  note: RMS LL
  note: Machine Disabled, Power sync on
  Prequest : Inport
  Fref : Inport  Port=2
  enabled : Inport  Port=3
  Vt : Inport  Port=4
  Vq : Inport  Port=5
  f_rotor : Inport  Port=6
  "LPF(DamperDecoupler) limited " : Subsystem
  Saturation1 : Saturate  UpperLimit=nominalFrequency+1  LowerLimit=nominalFrequency-1
  Scope1 : Scope  NumInputPorts=4
  Scope2 : Scope  NumInputPorts=3
  Sum : Sum  Inputs=|++
  Sum1 : Sum  Inputs=|+-
  Sum2 : Sum  Inputs=++|
  droop power limits : Saturate  UpperLimit=SRated  LowerLimit=-SRated
  k_droop : Gain  Gain=kDroop * SRated
  power request limits : Saturate  UpperLimit=SRated  LowerLimit=-SRated
  synchronizer : Subsystem
  power : Outport  VectorParamsAs1DForOutWhenUnconnected=on
  wires:
  power request limits/1 -> Scope1/1, Sum2/1
  droop power limits/1 -> Sum2/2
  synchronizer/1(p_sync_pu) -> Scope2/1, Sum/2  "p_sync"
  Vq/1 -> synchronizer/1(Vq), Scope2/2
  Prequest/1 -> power request limits/1
  k_droop/1 -> droop power limits/1
  Sum2/1 -> Scope1/2, "LPF(DamperDecoupler) limited "/1(In)
  "LPF(DamperDecoupler) limited "/1(Out) -> Scope1/3, Sum/1  "p_mechanical"
  Saturation1/1 -> Sum1/1
  f_rotor/1 -> Sum1/2
  Fref/1 -> Saturation1/1
  Sum/1 -> Scope1/4, power/1
  Sum1/1 -> k_droop/1
  Vt/1 -> synchronizer/2(Vt), Scope2/3
  enabled/1 -> synchronizer/3(machine_enabled)

== system My_gfm_battery_sil_2_Exciter_Dis/My Inverter Controller /My_machineModel_Other Exciter/impedance emulation ==
  v_emf : Inport
  enable : Inport  Port=2
  v_terminal : Inport  Port=3
  Constant : Constant  Value=0
  Integrator : Integrator
  Sum : Sum  Inputs=|+-
  Sum of Elements1 : Sum  Inputs=+
  Sum1 : Sum  Inputs=|+-
  Sum4 : Sum  Inputs=|+-
  Switch : Switch  Criteria=u2 > Threshold
  overLs : Gain  Gain=2*pi*60/(Xs * (VllRated^2/SRated))
  rN : Gain  Gain=rn*(VllRated^2/SRated)
  rs : Gain  Gain=rs*(VllRated^2/SRated)
  i_ref : Outport  VectorParamsAs1DForOutWhenUnconnected=on
  wires:
  enable/1 -> Switch/2
  Constant/1 -> Switch/3
  Sum/1 -> Switch/1
  Switch/1 -> Sum4/1
  v_terminal/1 -> Sum/2
  v_emf/1 -> Sum/1
  overLs/1 -> Integrator/1
  Sum of Elements1/1 -> rN/1
  Sum4/1 -> Sum1/1
  Sum1/1 -> overLs/1
  rN/1 -> Sum4/2
  rs/1 -> Sum1/2
  Integrator/1 -> Sum of Elements1/1, rs/1, i_ref/1  "i_ref"

== system My_gfm_battery_sil_2_Exciter_Dis/My Inverter Controller /My_machineModel_Other Exciter/power analyzer ==
  iac : Inport
  vac : Inport  Port=2
  Demux1 : Demux  Outputs=3
  Demux2 : Demux  Outputs=3
  Gain3 : Gain  Gain=1 / sqrt(3)
  Product{,1..3} (4 alike) : Product
  Sum of Elements : Sum  Inputs=+
  Sum2 : Sum  Inputs=|+-
  Sum3 : Sum  Inputs=|+-
  Sum4 : Sum  Inputs=|+-
  Sum5 : Sum  Inputs=+++
  P : Outport  VectorParamsAs1DForOutWhenUnconnected=on
  Q : Outport  Port=2  VectorParamsAs1DForOutWhenUnconnected=on
  wires:
  Product/1 -> Sum of Elements/1
  Sum of Elements/1 -> P/1  "P"
  Gain3/1 -> Q/1  "Q"
  Demux1/1 -> Product2/2  "ia"
  Demux2/1 -> Sum2/1, Sum4/2
  Sum2/1 -> Product1/1  "vab"
  Sum5/1 -> Gain3/1
  Sum3/1 -> Product2/1  "vbc"
  iac/1 -> Demux1/1, Product/1
  vac/1 -> Product/2, Demux2/1
  Demux1/2 -> Product3/2  "ib"
  Demux1/3 -> Product1/2  "ic"
  Demux2/3 -> Sum3/2, Sum4/1
  Demux2/2 -> Sum2/2, Sum3/1
  Product3/1 -> Sum5/2
  Sum4/1 -> Product3/1  "vca"
  Product2/1 -> Sum5/3
  Product1/1 -> Sum5/1

== system My_gfm_battery_sil_2_Exciter_Dis/My Inverter Controller /My_machineModel_Other Exciter/rotor model ==
  p_mechanical : Inport
  p_electrical : Inport  Port=2
  Constant : Constant  Value=nominalFrequency
  HPF (wDamperDecoupler) : TransferFcn  Commented=on  Numerator=[0.3 0]  Denominator=[0.3 1]
  HPF (wDamperDecoupler) 1 : Subsystem
  Integrator1 : Integrator  LimitOutput=on  UpperSaturationLimit=5  LowerSaturationLimit=-5
  Sum : Sum  Inputs=++|
  Sum2 : Sum  Inputs=|+-
  Sum3 : Sum  Inputs=|+-
  k_damp : Gain  Gain=kDamper*SRated
  k_inertia : Gain  Gain=(nominalFrequency/2)/(inertialConstant*SRated)
  oscillator_3ph : Subsystem
  osc[3] : Outport  VectorParamsAs1DForOutWhenUnconnected=on
  f_rotor : Outport  Port=2  VectorParamsAs1DForOutWhenUnconnected=on
  wires:
  Constant/1 -> Sum/1
  Sum/1 -> oscillator_3ph/1(f), f_rotor/1
  k_damp/1 -> Sum2/2
  Integrator1/1 -> HPF (wDamperDecoupler) 1/1(in), Sum/2
  p_mechanical/1 -> Sum3/1
  Sum3/1 -> Sum2/1
  p_electrical/1 -> Sum3/2
  HPF (wDamperDecoupler) 1/1(out) -> k_damp/1
  oscillator_3ph/1(osc[3]) -> osc[3]/1
  k_inertia/1 -> Integrator1/1
  Sum2/1 -> k_inertia/1

== system My_gfm_battery_sil_2_Exciter_Dis/My Inverter Controller /My_machineModel_Other Exciter/voltage analyzer ==
  osc[3] : Inport
  v_terminal : Inport  Port=2
  Complex to Magnitude-Angle : ComplexToMagnitudeAngle
  Complex to Real-Imag : ComplexToRealImag
  Conj : Math  Operator=conj  SaturateOnIntegerOverflow=on
  LPF : Subsystem
  "LPF " : Subsystem
  Product1 : Product
  Product2 : Product
  Real-Imag to Complex1 : RealImagToComplex
  Sum of Elements1 : Sum  Inputs=+
  Sum of Elements2 : Sum  Inputs=+
  Terminator : Terminator
  over_sqrt(3) : Gain  Gain=1/sqrt(3)
  over_sqrt(3)1 : Gain  Gain=1/sqrt(3)
  sqrt(2) : Gain  Gain=sqrt(2)
  Vd : Outport  VectorParamsAs1DForOutWhenUnconnected=on
  Vq : Outport  Port=2  VectorParamsAs1DForOutWhenUnconnected=on
  Vt_Mag : Outport  Port=3  VectorParamsAs1DForOutWhenUnconnected=on
  wires:
  "LPF "/1(Out) -> Real-Imag to Complex1/2, Vq/1  "Vq"
  osc[3]/1 -> Conj/1
  LPF/1(Out) -> Real-Imag to Complex1/1, Vd/1  "Vd"
  over_sqrt(3)1/1 -> LPF/1(In)
  over_sqrt(3)/1 -> "LPF "/1(In)
  Complex to Real-Imag/1 -> Product2/1
  Complex to Real-Imag/2 -> Product1/1
  Sum of Elements2/1 -> over_sqrt(3)1/1
  v_terminal/1 -> Product2/2, Product1/2
  Product1/1 -> Sum of Elements1/1
  Sum of Elements1/1 -> over_sqrt(3)/1
  sqrt(2)/1 -> Complex to Real-Imag/1
  Conj/1 -> sqrt(2)/1
  Product2/1 -> Sum of Elements2/1
  Complex to Magnitude-Angle/1 -> Vt_Mag/1  "Vt"
  Real-Imag to Complex1/1 -> Complex to Magnitude-Angle/1  "Vd"
  Complex to Magnitude-Angle/2 -> Terminator/1

== system My_gfm_battery_sil_2_Exciter_Dis/Plant controller (simplified example)/LVRT_foldback/LPF ==
  in : Inport
  1/0.01 : Gain  Gain=1/0.01
  Integrator : Integrator
  Sum3 : Sum  Inputs=|+-
  out : Outport  VectorParamsAs1DForOutWhenUnconnected=on
  wires:
  Integrator/1 -> out/1, Sum3/2
  Sum3/1 -> 1/0.01/1
  in/1 -> Sum3/1
  1/0.01/1 -> Integrator/1

== system My_gfm_battery_sil_2_Exciter_Dis/Plant controller (simplified example)/LVRT_foldback/assymmetric filter ==
  in : Inport
  Gain1 : Gain  Gain=1/0.01
  Integrator : Integrator
  Saturation1 : Saturate  UpperLimit=0.05 * 1  LowerLimit=-1 * 1
  Sum3 : Sum  Inputs=|+-
  out : Outport  VectorParamsAs1DForOutWhenUnconnected=on
  wires:
  Integrator/1 -> out/1, Sum3/2
  Sum3/1 -> Saturation1/1
  in/1 -> Sum3/1
  Gain1/1 -> Integrator/1
  Saturation1/1 -> Gain1/1

== system My_gfm_battery_sil_2_Exciter_Dis/Plant controller (simplified example)/Meter/PLL-analog ==
  note: cos x - j sin x
      | cos (x-120) - j (sin x -120)
      | cos (x+120) - j (sin x +120)
  note: cos x + j sin x
      | cos (x-120) + j (sin x -120)
      | cos (x+120) + j (sin x +120)
  note: -sin x
      |  -sin (x -120)
      |  -sin (x +120)
  note: cos x + j sin x
      | cos (x-120) + j (sin x -120)
      | cos (x+120) + j (sin x +120)
  ref : Inport
  Complex to Real-Imag : ComplexToRealImag
  Conj : Math  Operator=conj  SaturateOnIntegerOverflow=on
  Gain : Gain  Gain=3
  Gain2 : Gain  Gain=30
  Integrator : Integrator  LimitOutput=on  UpperSaturationLimit=5  LowerSaturationLimit=-5
  Product2 : Product
  Saturation : Saturate  UpperLimit=5  LowerLimit=-5
  Sum of Elements : Sum  Inputs=+
  Sum1 : Sum  Inputs=|++
  Sum2 : Sum  Inputs=|++
  Terminator : Terminator
  Transfer Fcn : TransferFcn  Denominator=[0.02 1]
  fnom : Constant  Value=60
  oscillator_3ph : Subsystem
  freq : Outport  VectorParamsAs1DForOutWhenUnconnected=on
  osc : Outport  Port=2  VectorParamsAs1DForOutWhenUnconnected=on
  wires:
  Gain2/1 -> Integrator/1
  Integrator/1 -> Sum2/2
  Sum2/1 -> Sum1/1
  fnom/1 -> Sum1/2
  Product2/1 -> Sum of Elements/1
  Transfer Fcn/1 -> Gain/1, Gain2/1
  Saturation/1 -> Sum2/1
  Gain/1 -> Saturation/1
  Sum1/1 -> oscillator_3ph/1(f), freq/1
  ref/1 -> Product2/1
  Sum of Elements/1 -> Transfer Fcn/1
  Conj/1 -> Complex to Real-Imag/1
  Complex to Real-Imag/1 -> Terminator/1
  Complex to Real-Imag/2 -> Product2/2
  oscillator_3ph/1(osc[3]) -> osc/1, Conj/1

== system My_gfm_battery_sil_2_Exciter_Dis/Plant controller (simplified example)/VoltVAr/LPF ==
  in : Inport
  1/0.05 : Gain  Gain=1/0.05
  Integrator : Integrator
  Sum3 : Sum  Inputs=|+-
  out : Outport  VectorParamsAs1DForOutWhenUnconnected=on
  wires:
  Integrator/1 -> out/1, Sum3/2
  Sum3/1 -> 1/0.05/1
  in/1 -> Sum3/1
  1/0.05/1 -> Integrator/1

== system My_gfm_battery_sil_2_Exciter_Dis/Plant controller (simplified example)/VoltVAr/LPF1 ==
  in : Inport
  1/0.05 : Gain  Gain=1/0.05
  1/0.1 : Gain
  Integrator : Integrator
  Saturation : Saturate  UpperLimit=inf  LowerLimit=0
  Saturation1 : Saturate  UpperLimit=0  LowerLimit=-inf
  Sum : Sum  Inputs=|++
  Sum3 : Sum  Inputs=|+-
  out : Outport  VectorParamsAs1DForOutWhenUnconnected=on
  wires:
  Integrator/1 -> out/1, Sum3/2
  Sum3/1 -> 1/0.1/1, 1/0.05/1
  in/1 -> Sum3/1
  1/0.05/1 -> Saturation/1
  Sum/1 -> Integrator/1
  1/0.1/1 -> Saturation1/1
  Saturation/1 -> Sum/1
  Saturation1/1 -> Sum/2

== system My_gfm_battery_sil_2_Exciter_Dis/My Inverter Controller /My_acMonitor_A/Analyzer_V/complex_LPF ==
  note: This was needed because Simulink complains when using transfer functions directly on arrays or complex numbers.
  In1 : Inport
  Complex to Real-Imag : ComplexToRealImag
  Gain2 : Gain  Gain=1/tau
  Gain3 : Gain  Gain=1/tau
  Integrator : Integrator
  Integrator1 : Integrator
  Real-Imag to Complex : RealImagToComplex
  Sum : Sum  Inputs=|+-
  Sum1 : Sum  Inputs=|+-
  Out1 : Outport  VectorParamsAs1DForOutWhenUnconnected=on
  wires:
  Real-Imag to Complex/1 -> Out1/1
  In1/1 -> Complex to Real-Imag/1
  Complex to Real-Imag/1 -> Sum/1
  Integrator/1 -> Real-Imag to Complex/1, Sum/2
  Sum1/1 -> Gain3/1
  Complex to Real-Imag/2 -> Sum1/1
  Gain2/1 -> Integrator/1
  Sum/1 -> Gain2/1
  Integrator1/1 -> Sum1/2, Real-Imag to Complex/2
  Gain3/1 -> Integrator1/1

== system My_gfm_battery_sil_2_Exciter_Dis/My Inverter Controller /My_acMonitor_A/Analyzer_V1/complex_LPF ==
  note: This was needed because Simulink complains when using transfer functions directly on arrays or complex numbers.
  In1 : Inport
  Complex to Real-Imag : ComplexToRealImag
  Gain2 : Gain  Gain=1/tau
  Gain3 : Gain  Gain=1/tau
  Integrator : Integrator
  Integrator1 : Integrator
  Real-Imag to Complex : RealImagToComplex
  Sum : Sum  Inputs=|+-
  Sum1 : Sum  Inputs=|+-
  Out1 : Outport  VectorParamsAs1DForOutWhenUnconnected=on
  wires:
  Real-Imag to Complex/1 -> Out1/1
  In1/1 -> Complex to Real-Imag/1
  Complex to Real-Imag/1 -> Sum/1
  Integrator/1 -> Real-Imag to Complex/1, Sum/2
  Sum1/1 -> Gain3/1
  Complex to Real-Imag/2 -> Sum1/1
  Gain2/1 -> Integrator/1
  Sum/1 -> Gain2/1
  Integrator1/1 -> Sum1/2, Real-Imag to Complex/2
  Gain3/1 -> Integrator1/1

== system My_gfm_battery_sil_2_Exciter_Dis/My Inverter Controller /My_acMonitor_A/PLL_3ph/oscillator_3ph ==
  f : Inport
  Cos : Trigonometry  Operator=cos
  Gain : Gain  Gain=2*pi
  Integrator : Integrator
  Real-Imag to Complex : RealImagToComplex
  Sin : Trigonometry
  Sum1 : Sum  Inputs=|++
  phase_shift : Constant  Value=[0 -1/3 -2/3]
  osc[3] : Outport  VectorParamsAs1DForOutWhenUnconnected=on
  wires:
  Sum1/1 -> Gain/1
  phase_shift/1 -> Sum1/2
  Sin/1 -> Real-Imag to Complex/2
  Integrator/1 -> Sum1/1
  Gain/1 -> Sin/1, Cos/1
  Cos/1 -> Real-Imag to Complex/1
  Real-Imag to Complex/1 -> osc[3]/1
  f/1 -> Integrator/1

== system My_gfm_battery_sil_2_Exciter_Dis/My Inverter Controller /My_circuit_controls_A/SOGI/Integrator1 ==
  In : Inport
  Ts : Inport  Port=2
  Delay1 : Delay  DelayLength=1
  Delay2 : Delay  DelayLength=1
  Delay3 : Delay  DelayLength=1
  Gain : Gain  Gain=1/12
  Gain1 : Gain  Gain=23
  Gain2 : Gain  Gain=16
  Gain3 : Gain  Gain=5
  Product : Product
  Sum : Sum  Inputs=|+-
  Sum1 : Sum  Inputs=|++
  Sum2 : Sum  Inputs=|++
  Out : Outport
  wires:
  Delay2/1 -> Gain2/1, Delay3/1
  Delay1/1 -> Sum2/2, Gain1/1, Delay2/1
  Delay3/1 -> Gain3/1
  Gain2/1 -> Sum/2
  Gain1/1 -> Sum/1
  Gain3/1 -> Sum1/2
  Sum/1 -> Sum1/1
  Gain/1 -> Sum2/1
  Sum2/1 -> Delay1/1
  Product/1 -> Gain/1
  Sum1/1 -> Out/1
  Ts/1 -> Product/2
  In/1 -> Product/1

== system My_gfm_battery_sil_2_Exciter_Dis/My Inverter Controller /My_circuit_controls_A/SOGI/Integrator3 ==
  In : Inport
  Ts : Inport  Port=2
  Delay1 : Delay  DelayLength=1
  Delay2 : Delay  DelayLength=1
  Delay3 : Delay  DelayLength=1
  Gain : Gain  Gain=1/12
  Gain1 : Gain  Gain=23
  Gain2 : Gain  Gain=16
  Gain3 : Gain  Gain=5
  Product : Product
  Sum : Sum  Inputs=|+-
  Sum1 : Sum  Inputs=|++
  Sum2 : Sum  Inputs=|++
  Out : Outport
  wires:
  Delay2/1 -> Gain2/1, Delay3/1
  Delay1/1 -> Sum2/2, Gain1/1, Delay2/1
  Delay3/1 -> Gain3/1
  Gain2/1 -> Sum/2
  Gain1/1 -> Sum/1
  Gain3/1 -> Sum1/2
  Sum/1 -> Sum1/1
  Gain/1 -> Sum2/1
  Sum2/1 -> Delay1/1
  Product/1 -> Gain/1
  Sum1/1 -> Out/1
  Ts/1 -> Product/2
  In/1 -> Product/1

== system My_gfm_battery_sil_2_Exciter_Dis/My Inverter Controller /My_circuit_controls_A/virtual damper/Damping HPF ==
  note: Forward integrator
  in : Inport
  Constant2 : Constant  Value=Ts
  Constant3 : Constant  Value=OmegaUp
  Constant4 : Constant  Value=OmegaDn
  Constant9 : Constant  Value=1/20000
  Delay : Delay  DelayLength=1  InitialCondition=0
  Gain : Gain  Gain=1/5
  Math Function : Math  Operator=reciprocal  SaturateOnIntegerOverflow=on
  MinMax : MinMax  Function=max  Inputs=2
  MinMax1 : MinMax  Inputs=2
  MinMax2 : MinMax  Inputs=2
  Product : Product
  Product1 : Product
  Product2 : Product
  Saturation : Saturate  UpperLimit=inf  LowerLimit=0
  Saturation1 : Saturate  UpperLimit=0  LowerLimit=-inf
  Sum : Sum  Inputs=|+-
  Sum1 : Sum  Inputs=|++
  Sum2 : Sum  Inputs=|++
  out : Outport
  wires:
  Gain/1 -> MinMax1/2, MinMax2/1
  [Ts] -> Product/1
  [Ts] -> Math Function/1
  Delay/1 -> Sum1/2, Sum/2
  MinMax1/1 -> [OmegaUp]
  Constant9/1 -> MinMax/2
  Sum/1 -> out/1, Product2/1, Product1/2
  Math Function/1 -> Gain/1
  Constant4/1 -> MinMax2/2
  Constant2/1 -> MinMax/1
  Saturation/1 -> Sum2/1
  Sum1/1 -> Delay/1
  Sum2/1 -> Product/2
  MinMax2/1 -> [OmegaDn]
  Product/1 -> Sum1/1
  [OmegaUp] -> Product1/1
  Constant3/1 -> MinMax1/1
  MinMax/1 -> [Ts]
  Product2/1 -> Saturation1/1
  in/1 -> Sum/1
  Product1/1 -> Saturation/1
  [OmegaDn] -> Product2/2
  Saturation1/1 -> Sum2/2

== system My_gfm_battery_sil_2_Exciter_Dis/My Inverter Controller /My_circuit_controls_A1/SOGI/Integrator1 ==
  In : Inport
  Ts : Inport  Port=2
  Delay1 : Delay  DelayLength=1
  Delay2 : Delay  DelayLength=1
  Delay3 : Delay  DelayLength=1
  Gain : Gain  Gain=1/12
  Gain1 : Gain  Gain=23
  Gain2 : Gain  Gain=16
  Gain3 : Gain  Gain=5
  Product : Product
  Sum : Sum  Inputs=|+-
  Sum1 : Sum  Inputs=|++
  Sum2 : Sum  Inputs=|++
  Out : Outport
  wires:
  Delay2/1 -> Gain2/1, Delay3/1
  Delay1/1 -> Sum2/2, Gain1/1, Delay2/1
  Delay3/1 -> Gain3/1
  Gain2/1 -> Sum/2
  Gain1/1 -> Sum/1
  Gain3/1 -> Sum1/2
  Sum/1 -> Sum1/1
  Gain/1 -> Sum2/1
  Sum2/1 -> Delay1/1
  Product/1 -> Gain/1
  Sum1/1 -> Out/1
  Ts/1 -> Product/2
  In/1 -> Product/1
